simulink library "sm_car_testrig_utilities_lib"  (R2025a)
settings: Solver=VariableStepAuto  StartTime=0.0  StopTime=10.0  RelTol=1e-3
undefined symbols (not defined in the file): Maneuver, tire_radius, Vehicle, Visual, X, Y, Z
libraries: sm_lib x31, nesl_utility x18, fl_lib x3, $bdroot x3, Tire_Utilities x2, Surface_Profile_Axle2_KnC x2, simulink x2
(part 1 of 2)
Description:
  | Copyright 2026 The MathWorks, Inc.
settings Model: Creator=smiller  LastModifiedBy=smiller
settings OptimizationCC: ReuseModelBlockBuffer=off
settings ModelReferenceCC: EnableRefExpFcnMdlSchedulingChecks=on
settings RTWCC: GPUComputeCapability=3.5

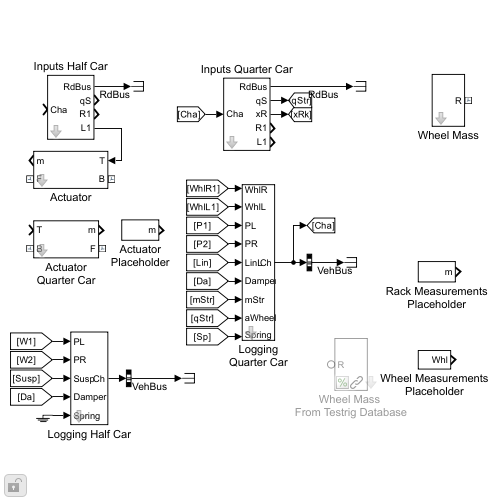
[thumbnail: Simulink's stored preview of the top-level diagram]
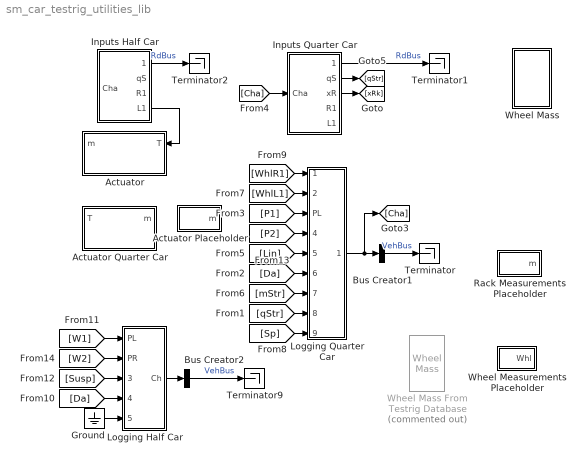
== system sm_car_testrig_utilities_lib ==
  Actuator : Subsystem  mask(KnC Actuator){tire_rad=tire_radius, xCPOffset=Maneuver.xCPOffset}
      mask prompts: tire_rad "Tire Radius (m)"; xCPOffset "xOffset from Contact Patch for force test (m)"
      mask help: Applies vertical motion to wheel center, permitting other DOFs to move freely. Can also apply force to wheel center, contact patch, and to a point behind the contact patch.
  Actuator Placeholder : Subsystem
  Actuator Quarter Car : Subsystem  mask{veh=Vehicle, xCPOffset=Maneuver.xCPOffset}
      mask prompts: veh "Vehicle (structure)"; xCPOffset "xOffset from Contact Patch for force test (m)"
      mask init:
      | tire_radii = sm_car_get_TireRadius(veh);
      | 
      | tire_radius = tire_radii(1);
      mask TypeOptions xCPOffset: Actuator/xCPOffset
  Bus Creator1 : BusCreator  Inputs=1
  Bus Creator2 : BusCreator  Inputs=1
  Ground : Ground
  Inputs Half Car : Subsystem  mask{popup_steering_input=On}
      mask prompts: popup_steering_input "Steering Input"
      mask init:
      | bh = gcb;
      | strIn = get_param(bh,'popup_steering_input');
      | set_param([bh '/Steering'], 'LabelModeActiveChoice',strIn);
      mask TypeOptions popup_steering_input: On | Off
  Inputs Quarter Car : Subsystem  mask{popup_steering_input=On}
      mask prompts: popup_steering_input "Steering Input"
      mask init:
      | bh = gcb;
      | strIn = get_param(bh,'popup_steering_input');
      | set_param([bh '/Steering'], 'LabelModeActiveChoice',strIn);
      mask TypeOptions popup_steering_input: On | Off
  Logging Quarter Car : Subsystem  mask(Logging Structure){}
      mask help: This subsystem takes logged signals and assembles them into a bus that has the same structure as the full vehicle model. This makes post-processing easier as the same scripts can be used.
      mask Display: disp(' ')
  Logging Half Car : Subsystem  mask(Logging Structure){}
      mask help: This subsystem takes logged signals and assembles them into a bus that has the same structure as the full vehicle model. This makes post-processing easier as the same scripts can be used.
      mask Display: disp(' ')
  Rack Measurements Placeholder : Subsystem
  Terminator{,1..2,9} (4 alike) : Terminator
  Wheel Mass : Subsystem  mask{tire_param=Vehicle.Chassis.TireA1.tirFile.Value}
      mask prompts: tire_param "Tire Parameters (structure)"
      mask init:
      | curblk = gcb;
      | 
      | %tireFile = evalin('base',get_param(curblk,'tire_param'));
      | %if(~contain(tire_param,'.tir'))
      | tireFile = tire_param;
      | if(contains(tireFile,'which'))
      |     tireFile = evalin('base',tireFile);
      | end
      | 
      | tirePar = simscape.multibody.tirread(tireFile);
      | 
      | tire_mass   = tirePar.INERTIA.MASS;
      | tire_radius = tirePar.DIMENSION.UNLOADED_RADIUS;
      | tire_width  = tirePar.DIMENSION.WIDTH;
  Wheel Mass From Testrig Database : $bdroot/Wheel Mass  Commented=on  tire_param=Vehicle.Chassis.TireA1
  Wheel Measurements Placeholder : Subsystem
  wires:
  [mStr] -> Logging Quarter Car/7(mStr)
  [Da] -> Logging Quarter Car/6(Damper)
  [Lin] -> Logging Quarter Car/5(LinL)
  [P2] -> Logging Quarter Car/4(PR)
  [qStr] -> Logging Quarter Car/8(aWheel)
  Inputs Quarter Car/2(qS) -> [qStr]
  Inputs Quarter Car/3(xR) -> [xRk]
  [Cha] -> Inputs Quarter Car/1(Cha)
  Logging Quarter Car/1(Ch) -> [Cha], Bus Creator1/1
  Bus Creator1/1 -> Terminator/1  "VehBus"
  Inputs Quarter Car/1(RdBus) -> Terminator1/1  "RdBus"
  [P1] -> Logging Quarter Car/3(PL)
  [WhlR1] -> Logging Quarter Car/1(WhlR)
  [WhlL1] -> Logging Quarter Car/2(WhlL)
  Inputs Half Car/1(RdBus) -> Terminator2/1  "RdBus"
  Logging Half Car/1(Ch) -> Bus Creator2/1
  Bus Creator2/1 -> Terminator9/1  "VehBus"
  [Sp] -> Logging Quarter Car/9(Spring)
  Ground/1 -> Logging Half Car/5(Spring)
  [Da] -> Logging Half Car/4(Damper)
  [Susp] -> Logging Half Car/3(Susp)
  [W2] -> Logging Half Car/2(PR)
  [W1] -> Logging Half Car/1(PL)
  Inputs Half Car/4(L1) -> Actuator/1(T)

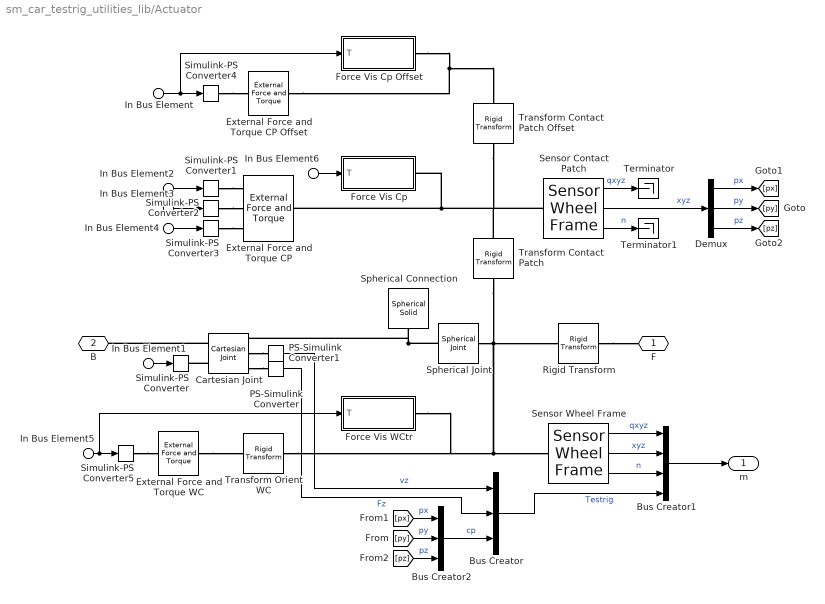
== system sm_car_testrig_utilities_lib/Actuator ==
  In Bus Element6 : Inport  PortName=T
  In Bus Element1 : Inport  PortName=T  Element=gz
  In Bus Element2 : Inport  PortName=T  Element=fcp.fx
  In Bus Element3 : Inport  PortName=T  Element=fcp.fy
  In Bus Element4 : Inport  PortName=T  Element=fcp.tz
  In Bus Element : Inport  PortName=T  Element=fcoy
  In Bus Element5 : Inport  PortName=T  Element=fwcx
  Bus Creator : BusCreator  Inputs=3
  Bus Creator1 : BusCreator  Inputs=4
  Bus Creator2 : BusCreator  Inputs=3
  Cartesian Joint : sm_lib/Joints/Cartesian Joint  JointMode=Normal  CompositeWrenchDir=FollowerOnBase  CompositeWrenchFrame=BaseFrame  SenseConstraintForce=off  SenseConstraintTorque=off  SenseTotalForce=off  SenseTotalTorque=off  PxPositionTargetSpecify=off  PxPositionTargetPriority=High  PxPositionTargetValue=0  PxPositionTargetValueUnits=m  PxVelocityTargetSpecify=off  PxVelocityTargetPriority=High  PxVelocityTargetValue=0  PxVelocityTargetValueUnits=m/s  PxEquilibriumPosition=0  PxEquilibriumPositionUnits=m  PxSpringStiffness=0  PxSpringStiffnessUnits=N/m  PxDampingCoefficient=0  PxDampingCoefficientUnits=N/(m/s)  PxLowerLimitSpecify=off  PxLowerLimitBound=-1  PxLowerLimitBoundUnits=m  PxLowerLimitStiffness=1e6  PxLowerLimitStiffnessUnits=N/m  PxLowerLimitDamping=1e3  PxLowerLimitDampingUnits=N/(m/s)  PxLowerLimitTransitionRegionWidth=1e-4  PxLowerLimitTransitionRegionWidthUnits=m  PxUpperLimitSpecify=off  PxUpperLimitBound=1  PxUpperLimitBoundUnits=m  PxUpperLimitStiffness=1e6  PxUpperLimitStiffnessUnits=N/m  PxUpperLimitDamping=1e3  PxUpperLimitDampingUnits=N/(m/s)  PxUpperLimitTransitionRegionWidth=1e-4  PxUpperLimitTransitionRegionWidthUnits=m  PxTorqueActuationMode=NoTorque  PxMotionActuationMode=ComputedMotion  PxSensePosition=off  PxSenseVelocity=off  PxSenseAcceleration=off  PxSenseTorqueForce=off  PxSenseLowerLimitTorqueForce=off  PxSenseUpperLimitTorqueForce=off  PyPositionTargetSpecify=off  PyPositionTargetPriority=High  PyPositionTargetValue=0  PyPositionTargetValueUnits=m  PyVelocityTargetSpecify=off  PyVelocityTargetPriority=High  PyVelocityTargetValue=0  PyVelocityTargetValueUnits=m/s  PyEquilibriumPosition=0  PyEquilibriumPositionUnits=m  PySpringStiffness=0  PySpringStiffnessUnits=N/m  PyDampingCoefficient=0  PyDampingCoefficientUnits=N/(m/s)  PyLowerLimitSpecify=off  PyLowerLimitBound=-1  PyLowerLimitBoundUnits=m  PyLowerLimitStiffness=1e6  PyLowerLimitStiffnessUnits=N/m  PyLowerLimitDamping=1e3  PyLowerLimitDampingUnits=N/(m/s)  PyLowerLimitTransitionRegionWidth=1e-4  PyLowerLimitTransitionRegionWidthUnits=m  PyUpperLimitSpecify=off  PyUpperLimitBound=1  PyUpperLimitBoundUnits=m  PyUpperLimitStiffness=1e6  PyUpperLimitStiffnessUnits=N/m  PyUpperLimitDamping=1e3  PyUpperLimitDampingUnits=N/(m/s)  PyUpperLimitTransitionRegionWidth=1e-4  PyUpperLimitTransitionRegionWidthUnits=m  PyTorqueActuationMode=NoTorque  PyMotionActuationMode=ComputedMotion  PySensePosition=off  PySenseVelocity=off  PySenseAcceleration=off  PySenseTorqueForce=off  PySenseLowerLimitTorqueForce=off  PySenseUpperLimitTorqueForce=off  PzPositionTargetSpecify=off  PzPositionTargetPriority=High  PzPositionTargetValue=0  PzPositionTargetValueUnits=m  PzVelocityTargetSpecify=off  PzVelocityTargetPriority=High  PzVelocityTargetValue=0  PzVelocityTargetValueUnits=m/s  PzEquilibriumPosition=0  PzEquilibriumPositionUnits=m  PzSpringStiffness=0  PzSpringStiffnessUnits=N/m  PzDampingCoefficient=0  PzDampingCoefficientUnits=N/(m/s)  PzLowerLimitSpecify=off  PzLowerLimitBound=-1  PzLowerLimitBoundUnits=m  PzLowerLimitStiffness=1e6  PzLowerLimitStiffnessUnits=N/m  PzLowerLimitDamping=1e3  PzLowerLimitDampingUnits=N/(m/s)  PzLowerLimitTransitionRegionWidth=1e-4  PzLowerLimitTransitionRegionWidthUnits=m  PzUpperLimitSpecify=off  PzUpperLimitBound=1  PzUpperLimitBoundUnits=m  PzUpperLimitStiffness=1e6  PzUpperLimitStiffnessUnits=N/m  PzUpperLimitDamping=1e3  PzUpperLimitDampingUnits=N/(m/s)  PzUpperLimitTransitionRegionWidth=1e-4  PzUpperLimitTransitionRegionWidthUnits=m  PzTorqueActuationMode=ComputedTorque  PzMotionActuationMode=InputMotion  PzSensePosition=off  PzSenseVelocity=on  PzSenseAcceleration=off  PzSenseTorqueForce=on  PzSenseLowerLimitTorqueForce=off  PzSenseUpperLimitTorqueForce=off
  Demux : Demux  Outputs=3
  External Force and Torque WC : sm_lib/Forces and Torques/External Force and Torque  EnableForceX=off  EnableForceY=on  EnableForceZ=off  EnableForce=off  ForceResolutionFrame=World  EnableTorqueX=off  EnableTorqueY=off  EnableTorqueZ=off  EnableTorque=off  TorqueResolutionFrame=World
  External Force and Torque CP : sm_lib/Forces and Torques/External Force and Torque  EnableForceX=on  EnableForceY=on  EnableForceZ=off  EnableForce=off  ForceResolutionFrame=World  EnableTorqueX=off  EnableTorqueY=off  EnableTorqueZ=on  EnableTorque=off  TorqueResolutionFrame=World
  External Force and Torque CP Offset : sm_lib/Forces and Torques/External Force and Torque  EnableForceX=off  EnableForceY=on  EnableForceZ=off  EnableForce=off  ForceResolutionFrame=World  EnableTorqueX=off  EnableTorqueY=off  EnableTorqueZ=off  EnableTorque=off  TorqueResolutionFrame=World
  Force Vis Cp : Subsystem  mask(Force and Torque Visualization){fcyl_opc=0.2, fcyl_clr=[1 0 0], fcyl_rad=0.02, fcyl_len=0.8, tcyl_rad=0.25, tcyl_clrn=[0.3922 0.8314 0.07451], max_fx=max(Maneuver.PostL1.fx.Value), max_fy=max(Maneuver.PostL1.fy.Value), max_tz=max(Maneuver.PostL1.tz.Value)}
      mask prompts: fcyl_opc "Opacity (0-1)"; fcyl_clr "Color [RGB]"; fcyl_rad "Radius (m)"; fcyl_len "Max Length (m)"; tcyl_rad "Max Radius (m)"; tcyl_clrn "Color for negative [RGB]"; max_fx "Max Fx (N)"; max_fy "Max Fy (N)"; max_tz "Max Tz (N)"
      mask help: Provides visual element for force and torque. Force visualization extends in direction along which force is applied. Torque visualization uses alternate color for opposite sign.
      mask DialogControl cont_fcyl Prompt: Force Cylinders
      mask DialogControl cont_trqcyl Prompt: Torque Cylinders
      mask DialogControl cont_fmax Prompt: Force/Torque Magnitudes
  Force Vis Cp Offset : Subsystem  mask(Force Visualization){fcyl_opc=0.2, fcyl_clr=[1 0 0], fcyl_rad=0.02, fcyl_len=0.8, tcyl_rad=0.25, tcyl_clrn=[0.3922 0.8314 0.07451], fy_max=max(Maneuver.PostL1.fcoy.Value)}
      mask prompts: fcyl_opc "Opacity (0-1)"; fcyl_clr "Color [RGB]"; fcyl_rad "Radius (m)"; fcyl_len "Max Length (m)"; tcyl_rad "Max Radius (m)"; tcyl_clrn "Color for negative [RGB]"; fy_max "Max Fx (N)"
      mask help: Provides visual element for force. Extends in direction along which force is applied.
      mask DialogControl cont_fcyl Prompt: Force Cylinders
      mask DialogControl cont_trqcyl Prompt: Torque Cylinders
      mask DialogControl cont_fmx Prompt: Force Magnitudes
  Force Vis WCtr : Subsystem  mask(Force Visualization){fcyl_opc=0.2, fcyl_clr=[1 0 0], fcyl_rad=0.02, fcyl_len=0.8, max_fx=max(Maneuver.PostL1.fwcx.Value)}
      mask prompts: fcyl_opc "Opacity (0-1)"; fcyl_clr "Color [RGB]"; fcyl_rad "Radius (m)"; fcyl_len "Max Length (m)"; max_fx "Max Fx(N)"
      mask help: Provides visual element for force. Extends in direction along which force is applied.
      mask DialogControl cont_fcyl Prompt: Force Cylinders
      mask DialogControl cont_fmax Prompt: Force Magnitudes
  PS-Simulink Converter : nesl_utility/PS-Simulink Converter  PhysicalDomain=network_engine_domain  SubClassName=ps_output  LeftPortType=input  RightPortType=output  PseudoPeriodic=off  Frequencies=[]  VectorFormat=1-D array  Unit=1  AffineConversion=off
  PS-Simulink Converter1 : nesl_utility/PS-Simulink Converter  PhysicalDomain=network_engine_domain  SubClassName=ps_output  LeftPortType=input  RightPortType=output  PseudoPeriodic=off  Frequencies=[]  VectorFormat=1-D array  Unit=1  AffineConversion=off
  Rigid Transform : sm_lib/Frames and Transforms/Rigid Transform  RotationMethod=StandardAxis  FollAlignAxisA=+X  BaseAlignAxisA=+Y  FollAlignAxisB=+Y  BaseAlignAxisB=+Z  RotationStandardAxis=+X  RotationAngle=-90  RotationAngleUnits=deg  RotationArbitraryAxis=[0 0 1]  RotationSequenceAxes=FollowerAxes  RotationSequence=XYX  RotationSequenceAngles=[0 0 0]  RotationSequenceAnglesUnits=deg  RotationMatrix=[1 0 0; 0 1 0; 0 0 1]  Quaternion=[1 0 0 0]  TranslationMethod=None  TranslationCartesianOffset=[0 0 0]  TranslationCartesianOffsetUnits=m  TranslationStandardAxis=+Z  TranslationStandardOffset=0  TranslationStandardOffsetUnits=m  TranslationROffset=0  TranslationROffsetUnits=m  TranslationThetaOffset=0  TranslationThetaOffsetUnits=deg  TranslationZOffset=0  TranslationZOffsetUnits=m
  Sensor Contact Patch : Tire_Utilities/Sensor Wheel Frame  SystemSampleTime=-1  VariantActivationTime=update diagram  EmptyChoice=off  PassThrough=off  PassThroughVariantControl=(default)  EmptyChoiceVariantControl=(default)  AllowFlexibleInterface=on  Latency=0  AutoFrameSizeCalculation=off
  Sensor Wheel Frame : Tire_Utilities/Sensor Wheel Frame  SystemSampleTime=-1  VariantActivationTime=update diagram  EmptyChoice=off  PassThrough=off  PassThroughVariantControl=(default)  EmptyChoiceVariantControl=(default)  AllowFlexibleInterface=on  Latency=0  AutoFrameSizeCalculation=off
  Simulink-PS Converter : nesl_utility/Simulink-PS Converter  PhysicalDomain=network_engine_domain  SubClassName=ps_input  LeftPortType=input  RightPortType=output  PseudoPeriodic=off  Frequencies=[]  NoiseDistribution=none  NoiseParameters=[]  Unit=m  AffineConversion=off  FilteringAndDerivatives=filter  SimscapeFilterOrder=2  InputFilterTimeConstant=0.1  UdotUserProvided=0
  Simulink-PS Converter{1..5} (5 alike) : nesl_utility/Simulink-PS Converter  PhysicalDomain=network_engine_domain  SubClassName=ps_input  LeftPortType=input  RightPortType=output  PseudoPeriodic=off  Frequencies=[]  NoiseDistribution=none  NoiseParameters=[]  Unit=1  AffineConversion=off  FilteringAndDerivatives=provide  SimscapeFilterOrder=1  InputFilterTimeConstant=0.001  UdotUserProvided=0
  Spherical Connection : sm_lib/Body Elements/Spherical Solid  SphereRadius=Visual.hp.rad*1.5  SphereRadiusUnits=m  ExportEntireGeometry=off  InertiaType=CalculateFromGeometry  BasedOnType=Density  Density=1000  DensityUnits=kg/m^3  Mass=1  MassUnits=kg  CenterOfMass=[0 0 0]  CenterOfMassUnits=m  MomentsOfInertia=[1 1 1]  MomentsOfInertiaUnits=kg*m^2  ProductsOfInertia=[0 0 0]  ProductsOfInertiaUnits=kg*m^2  GraphicType=FromGeometry  MarkerShape=Sphere  MarkerSize=10  GraphicVisPropType=SimpleVisualProperties  GraphicDiffuseColor=[0.2 0.2 1.0]  GraphicOpacity=0.5  GraphicSpecularColor=[0.5 0.5 0.5 1.0]  GraphicAmbientColor=[0.15 0.15 0.15 1.0]  GraphicEmissiveColor=[0.0 0.0 0.0 1.0]  GraphicShininess=75  DoExposeReferenceFrame=on  SerializedFrames=<Frames/>
  Spherical Joint : sm_lib/Joints/Spherical Joint  JointMode=Normal  CompositeWrenchDir=FollowerOnBase  CompositeWrenchFrame=BaseFrame  SenseConstraintForce=off  SenseConstraintTorque=off  SenseTotalForce=off  SenseTotalTorque=off  PositionTargetSpecify=off  PositionTargetPriority=High  PositionTargetRotationMethod=None  PositionTargetFollAlignAxisA=+X  PositionTargetBaseAlignAxisA=+Y  PositionTargetFollAlignAxisB=+Y  PositionTargetBaseAlignAxisB=+Z  PositionTargetRotationStandardAxis=+Z  PositionTargetRotationAngle=0.0  PositionTargetRotationAngleUnits=deg  PositionTargetRotationArbitraryAxis=[0 0 1]  PositionTargetRotationSequenceAxes=FollowerAxes  PositionTargetRotationSequence=XYX  PositionTargetRotationSequenceAngles=[0 0 0]  PositionTargetRotationSequenceAnglesUnits=deg  PositionTargetRotationMatrix=[1 0 0; 0 1 0; 0 0 1]  PositionTargetQuaternion=[1 0 0 0]  VelocityTargetSpecify=off  VelocityTargetPriority=High  VelocityTargetValue=[0 0 0]  VelocityTargetValueUnits=deg/s  VelocityTargetInFollowerFrame=on  EqPosRotationMethod=None  EqPosFollAlignAxisA=+X  EqPosBaseAlignAxisA=+Y  EqPosFollAlignAxisB=+Y  EqPosBaseAlignAxisB=+Z  EqPosRotationStandardAxis=+Z  EqPosRotationAngle=0.0  EqPosRotationAngleUnits=deg  EqPosRotationArbitraryAxis=[0 0 1]  EqPosRotationSequenceAxes=FollowerAxes  EqPosRotationSequence=XYX  EqPosRotationSequenceAngles=[0 0 0]  EqPosRotationSequenceAnglesUnits=deg  EqPosRotationMatrix=[1 0 0; 0 1 0; 0 0 1]  EqPosQuaternion=[1 0 0 0]  SpringStiffness=0  SpringStiffnessUnits=N*m/deg  DampingCoefficient=0  DampingCoefficientUnits=N*m/(deg/s)  LowerLimitSpecify=off  LowerLimitBound=15  LowerLimitBoundUnits=deg  LowerLimitStiffness=1e4  LowerLimitStiffnessUnits=N*m/deg  LowerLimitDamping=10  LowerLimitDampingUnits=N*m/(deg/s)  LowerLimitTransitionRegionWidth=0.1  LowerLimitTransitionRegionWidthUnits=deg  UpperLimitSpecify=off  UpperLimitBound=45  UpperLimitBoundUnits=deg  UpperLimitStiffness=1e4  UpperLimitStiffnessUnits=N*m/deg  UpperLimitDamping=10  UpperLimitDampingUnits=N*m/(deg/s)  UpperLimitTransitionRegionWidth=0.1  UpperLimitTransitionRegionWidthUnits=deg  TorqueActuationMode=NoTorque  ActuateTorqueX=off  ActuateTorqueY=off  ActuateTorqueZ=off  ActuateTorque=off  ActuationFrame=BaseFrame  SensePosition=off  SenseVelocityX=off  SenseVelocityY=off  SenseVelocityZ=off  SenseVelocity=off  SenseAccelerationX=off  SenseAccelerationY=off  SenseAccelerationZ=off  SenseAcceleration=off  SenseLowerLimitTorqueMag=off  SenseUpperLimitTorqueMag=off  SensingFrame=BaseFrame
  Terminator : Terminator
  Terminator1 : Terminator
  Transform Contact Patch : sm_lib/Frames and Transforms/Rigid Transform  RotationMethod=None  FollAlignAxisA=+X  BaseAlignAxisA=+Y  FollAlignAxisB=+Y  BaseAlignAxisB=+Z  RotationStandardAxis=+X  RotationAngle=90  RotationAngleUnits=deg  RotationArbitraryAxis=[0 0 1]  RotationSequenceAxes=FollowerAxes  RotationSequence=XYX  RotationSequenceAngles=[0 0 0]  RotationSequenceAnglesUnits=deg  RotationMatrix=[1 0 0; 0 1 0; 0 0 1]  Quaternion=[1 0 0 0]  TranslationMethod=Cartesian  TranslationCartesianOffset=[0 0 -tire_rad]  TranslationCartesianOffsetUnits=m  TranslationStandardAxis=+Z  TranslationStandardOffset=0  TranslationStandardOffsetUnits=m  TranslationROffset=0  TranslationROffsetUnits=m  TranslationThetaOffset=0  TranslationThetaOffsetUnits=deg  TranslationZOffset=0  TranslationZOffsetUnits=m
  Transform Contact Patch Offset : sm_lib/Frames and Transforms/Rigid Transform  RotationMethod=None  FollAlignAxisA=+X  BaseAlignAxisA=+Y  FollAlignAxisB=+Y  BaseAlignAxisB=+Z  RotationStandardAxis=+X  RotationAngle=90  RotationAngleUnits=deg  RotationArbitraryAxis=[0 0 1]  RotationSequenceAxes=FollowerAxes  RotationSequence=XYX  RotationSequenceAngles=[0 0 0]  RotationSequenceAnglesUnits=deg  RotationMatrix=[1 0 0; 0 1 0; 0 0 1]  Quaternion=[1 0 0 0]  TranslationMethod=Cartesian  TranslationCartesianOffset=[xCPOffset 0 0]  TranslationCartesianOffsetUnits=m  TranslationStandardAxis=+Z  TranslationStandardOffset=0  TranslationStandardOffsetUnits=m  TranslationROffset=0  TranslationROffsetUnits=m  TranslationThetaOffset=0  TranslationThetaOffsetUnits=deg  TranslationZOffset=0  TranslationZOffsetUnits=m
  Transform Orient WC : sm_lib/Frames and Transforms/Rigid Transform  RotationMethod=StandardAxis  FollAlignAxisA=+X  BaseAlignAxisA=+Y  FollAlignAxisB=+Y  BaseAlignAxisB=+Z  RotationStandardAxis=+X  RotationAngle=90  RotationAngleUnits=deg  RotationArbitraryAxis=[0 0 1]  RotationSequenceAxes=FollowerAxes  RotationSequence=XYX  RotationSequenceAngles=[0 0 0]  RotationSequenceAnglesUnits=deg  RotationMatrix=[1 0 0; 0 1 0; 0 0 1]  Quaternion=[1 0 0 0]  TranslationMethod=Cartesian  TranslationCartesianOffset=[0 0 0]  TranslationCartesianOffsetUnits=m  TranslationStandardAxis=+Z  TranslationStandardOffset=0  TranslationStandardOffsetUnits=m  TranslationROffset=0  TranslationROffsetUnits=m  TranslationThetaOffset=0  TranslationThetaOffsetUnits=deg  TranslationZOffset=0  TranslationZOffsetUnits=m
  F : PMIOPort  Side=Right
  B : PMIOPort  Port=2  Side=Left
  m : Outport  VectorParamsAs1DForOutWhenUnconnected=off
  wires:
  In Bus Element1/1 -> Simulink-PS Converter/1
  In Bus Element3/1 -> Simulink-PS Converter2/1
  Demux/2 -> [py]  "py"
  In Bus Element4/1 -> Simulink-PS Converter3/1
  Sensor Contact Patch/2 -> Demux/1  "xyz"
  Sensor Contact Patch/1 -> Terminator/1  "qxyz"
  In Bus Element2/1 -> Simulink-PS Converter1/1
  Sensor Contact Patch/3 -> Terminator1/1  "n"
  Sensor Wheel Frame/2 -> Bus Creator1/2  "xyz"
  Sensor Wheel Frame/1 -> Bus Creator1/1  "qxyz"
  Bus Creator/1 -> Bus Creator1/4  "Testrig"
  Bus Creator1/1 -> m/1
  PS-Simulink Converter/1 -> Bus Creator/2  "Fz"
  Sensor Wheel Frame/3 -> Bus Creator1/3  "n"
  [py] -> Bus Creator2/2  "py"
  Demux/1 -> [px]  "px"
  [px] -> Bus Creator2/1  "px"
  In Bus Element/1 -> Force Vis Cp Offset/1(T), Simulink-PS Converter4/1
  In Bus Element5/1 -> Force Vis WCtr/1(T), Simulink-PS Converter5/1
  In Bus Element6/1 -> Force Vis Cp/1(T)
  PS-Simulink Converter1/1 -> Bus Creator/1  "vz"
  Demux/3 -> [pz]  "pz"
  [pz] -> Bus Creator2/3  "pz"
  Bus Creator2/1 -> Bus Creator/3  "cp"
  connections:
  Rigid Transform/RConn1 -- F/RConn1
  Spherical Joint/LConn1 -- Cartesian Joint/RConn1 -- Spherical Connection/RConn1
  Spherical Joint/RConn1 -- Force Vis WCtr/RConn1 -- Transform Orient WC/LConn1 -- Sensor Wheel Frame/LConn1 -- Transform Contact Patch/LConn1 -- Rigid Transform/LConn1
  Cartesian Joint/LConn1 -- B/RConn1
  Cartesian Joint/LConn2 -- Simulink-PS Converter/RConn1
  Cartesian Joint/RConn3 -- PS-Simulink Converter/LConn1
  Transform Contact Patch Offset/LConn1 -- Sensor Contact Patch/LConn1 -- Transform Contact Patch/RConn1 -- External Force and Torque CP/RConn1 -- Force Vis Cp/RConn1
  Simulink-PS Converter1/RConn1 -- External Force and Torque CP/LConn1
  Simulink-PS Converter3/RConn1 -- External Force and Torque CP/LConn3
  Simulink-PS Converter2/RConn1 -- External Force and Torque CP/LConn2
  External Force and Torque CP Offset/RConn1 -- Force Vis Cp Offset/RConn1 -- Transform Contact Patch Offset/RConn1
  Simulink-PS Converter4/RConn1 -- External Force and Torque CP Offset/LConn1
  Simulink-PS Converter5/RConn1 -- External Force and Torque WC/LConn1
  External Force and Torque WC/RConn1 -- Transform Orient WC/RConn1
  Cartesian Joint/RConn2 -- PS-Simulink Converter1/LConn1

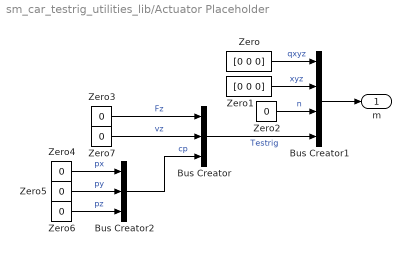
== system sm_car_testrig_utilities_lib/Actuator Placeholder ==
  Bus Creator : BusCreator  Inputs=3
  Bus Creator1 : BusCreator  Inputs=4
  Bus Creator2 : BusCreator  Inputs=3
  Zero : Constant  Value=[0 0 0]  OutDataTypeStr=Inherit: Inherit via back propagation
  Zero1 : Constant  Value=[0 0 0]  OutDataTypeStr=Inherit: Inherit via back propagation
  Zero{2..7} (6 alike) : Constant  Value=0  OutDataTypeStr=Inherit: Inherit via back propagation
  m : Outport
  wires:
  Zero4/1 -> Bus Creator2/1  "px"
  Zero1/1 -> Bus Creator1/2  "xyz"
  Zero2/1 -> Bus Creator1/3  "n"
  Zero/1 -> Bus Creator1/1  "qxyz"
  Zero3/1 -> Bus Creator/1  "Fz"
  Zero5/1 -> Bus Creator2/2  "py"
  Bus Creator/1 -> Bus Creator1/4  "Testrig"
  Bus Creator1/1 -> m/1
  Zero6/1 -> Bus Creator2/3  "pz"
  Bus Creator2/1 -> Bus Creator/3  "cp"
  Zero7/1 -> Bus Creator/2  "vz"

== system sm_car_testrig_utilities_lib/Actuator Quarter Car ==
  T : Inport
  Actuator : $bdroot/Actuator  tire_rad=tire_radius  xCPOffset=xCPOffset
  F : PMIOPort  Side=Right
  B : PMIOPort  Port=2  Side=Left
  m : Outport
  wires:
  Actuator/1 -> m/1
  T/1 -> Actuator/1
  connections:
  Actuator/LConn1 -- B/RConn1
  Actuator/RConn1 -- F/RConn1

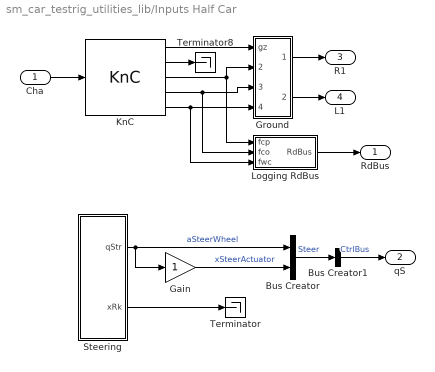
== system sm_car_testrig_utilities_lib/Inputs Half Car ==
  Cha : Inport
  Bus Creator : BusCreator  Inputs=2
  Bus Creator1 : BusCreator  Inputs=1
  Gain : Gain
  Ground : Subsystem
  KnC : Surface_Profile_Axle2_KnC/KnC  SystemSampleTime=-1  VariantControl=KnC  VariantActivationTime=update diagram  EmptyChoice=off  PassThrough=off  PassThroughVariantControl=(default)  EmptyChoiceVariantControl=(default)  AllowFlexibleInterface=on  Latency=0  AutoFrameSizeCalculation=off
  Logging RdBus : Subsystem
  Steering : Subsystem  Variant=on  VariantControlMode=label  VariantControl=Choice  LabelModeActiveChoice=On
  Terminator : Terminator
  Terminator8 : Terminator
  RdBus : Outport
  qS : Outport  Port=2
  R1 : Outport  Port=3
  L1 : Outport  Port=4
  wires:
  Logging RdBus/1(RdBus) -> RdBus/1
  Steering/2(xRk) -> Terminator/1
  Steering/1(qStr) -> Gain/1, Bus Creator/1  "aSteerWheel"
  Ground/1(R1) -> R1/1
  Cha/1 -> KnC/1
  KnC/1 -> Ground/1(gz)
  Ground/2(L1) -> L1/1
  KnC/3 -> Logging RdBus/1(fcp), Ground/2(fcp)
  KnC/2 -> Terminator8/1
  Bus Creator1/1 -> qS/1  "CtrlBus"
  Bus Creator/1 -> Bus Creator1/1  "Steer"
  KnC/4 -> Logging RdBus/2(fco), Ground/3(fco)
  KnC/5 -> Logging RdBus/3(fwc), Ground/4(fwc)
  Gain/1 -> Bus Creator/2  "xSteerActuator"

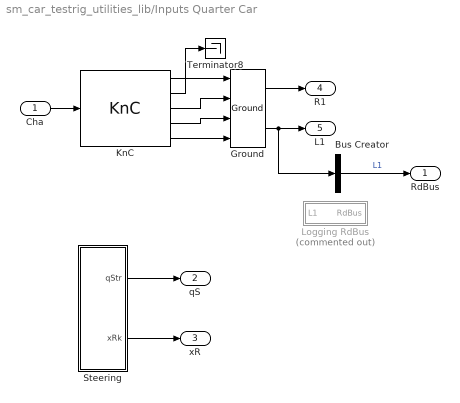
== system sm_car_testrig_utilities_lib/Inputs Quarter Car ==
  Cha : Inport
  Bus Creator : BusCreator  Inputs=1
  Ground : $bdroot/Inputs Half Car/Ground  SystemSampleTime=-1  VariantActivationTime=update diagram  EmptyChoice=off  PassThrough=off  PassThroughVariantControl=(default)  EmptyChoiceVariantControl=(default)  AllowFlexibleInterface=on  Latency=0  AutoFrameSizeCalculation=off
  KnC : Surface_Profile_Axle2_KnC/KnC  SystemSampleTime=-1  VariantControl=KnC  VariantActivationTime=update diagram  EmptyChoice=off  PassThrough=off  PassThroughVariantControl=(default)  EmptyChoiceVariantControl=(default)  AllowFlexibleInterface=on  Latency=0  AutoFrameSizeCalculation=off
  Logging RdBus : Subsystem  Commented=on
  Steering : Subsystem  Variant=on  VariantControlMode=label  VariantControl=Choice  LabelModeActiveChoice=On
  Terminator8 : Terminator
  RdBus : Outport
  qS : Outport  Port=2
  xR : Outport  Port=3
  R1 : Outport  Port=4
  L1 : Outport  Port=5
  wires:
  KnC/2 -> Terminator8/1
  KnC/3 -> Ground/2
  KnC/1 -> Ground/1
  Cha/1 -> KnC/1
  Ground/1 -> R1/1
  Steering/1(qStr) -> qS/1
  Steering/2(xRk) -> xR/1
  Ground/2 -> Bus Creator/1, L1/1
  KnC/4 -> Ground/3
  KnC/5 -> Ground/4
  Bus Creator/1 -> RdBus/1  "L1"

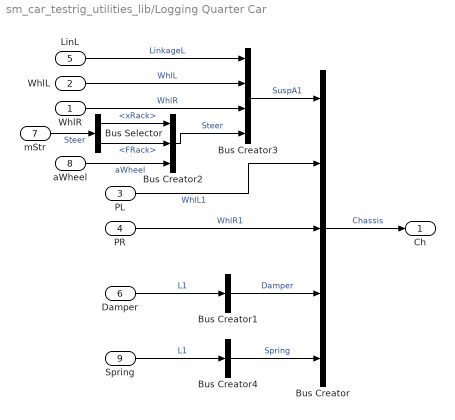
== system sm_car_testrig_utilities_lib/Logging Quarter Car ==
  WhlR : Inport
  WhlL : Inport  Port=2
  PL : Inport  Port=3
  PR : Inport  Port=4
  LinL : Inport  Port=5
  Damper : Inport  Port=6
  mStr : Inport  Port=7
  aWheel : Inport  Port=8
  Spring : Inport  Port=9
  Bus Creator : BusCreator  Inputs=5
  Bus Creator1 : BusCreator  Inputs=1
  Bus Creator2 : BusCreator  Inputs=3
  Bus Creator3 : BusCreator  Inputs=4
  Bus Creator4 : BusCreator  Inputs=1
  Bus Selector : BusSelector  OutputSignals=xRack,FRack
  Ch : Outport
  wires:
  Bus Selector/2 -> Bus Creator2/2  "<FRack>"
  Bus Selector/1 -> Bus Creator2/1  "<xRack>"
  mStr/1 -> Bus Selector/1  "Steer"
  PR/1 -> Bus Creator/3  "WhlR1"
  WhlR/1 -> Bus Creator3/3  "WhlR"
  PL/1 -> Bus Creator/2  "WhlL1"
  Bus Creator3/1 -> Bus Creator/1  "SuspA1"
  Bus Creator/1 -> Ch/1  "Chassis"
  LinL/1 -> Bus Creator3/1  "LinkageL"
  WhlL/1 -> Bus Creator3/2  "WhlL"
  Damper/1 -> Bus Creator1/1  "L1"
  Bus Creator2/1 -> Bus Creator3/4  "Steer"
  Bus Creator1/1 -> Bus Creator/4  "Damper"
  aWheel/1 -> Bus Creator2/3  "aWheel"
  Spring/1 -> Bus Creator4/1  "L1"
  Bus Creator4/1 -> Bus Creator/5  "Spring"

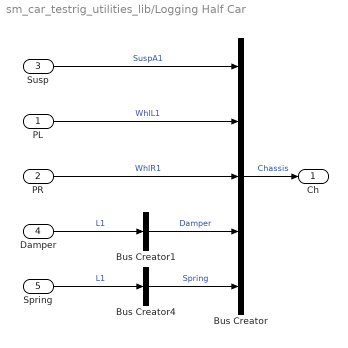
== system sm_car_testrig_utilities_lib/Logging Half Car ==
  PL : Inport
  PR : Inport  Port=2
  Susp : Inport  Port=3
  Damper : Inport  Port=4
  Spring : Inport  Port=5
  Bus Creator : BusCreator  Inputs=5
  Bus Creator1 : BusCreator  Inputs=1
  Bus Creator4 : BusCreator  Inputs=1
  Ch : Outport
  wires:
  PR/1 -> Bus Creator/3  "WhlR1"
  Bus Creator4/1 -> Bus Creator/5  "Spring"
  Spring/1 -> Bus Creator4/1  "L1"
  Bus Creator1/1 -> Bus Creator/4  "Damper"
  Damper/1 -> Bus Creator1/1  "L1"
  Bus Creator/1 -> Ch/1  "Chassis"
  Susp/1 -> Bus Creator/1  "SuspA1"
  PL/1 -> Bus Creator/2  "WhlL1"

== system sm_car_testrig_utilities_lib/Rack Measurements Placeholder ==
  Bus Creator2 : BusCreator  Inputs=2
  Zero3 : Constant  Value=0  OutDataTypeStr=Inherit: Inherit via back propagation
  Zero4 : Constant  Value=0  OutDataTypeStr=Inherit: Inherit via back propagation
  m : Outport
  wires:
  Bus Creator2/1 -> m/1
  Zero4/1 -> Bus Creator2/2  "FRack"
  Zero3/1 -> Bus Creator2/1  "xRack"

== system sm_car_testrig_utilities_lib/Wheel Mass ==
  Wheel Mass : sm_lib/Body Elements/Cylindrical Solid  CylinderRadius=tire_radius  CylinderRadiusUnits=m  CylinderLength=tire_width  CylinderLengthUnits=m  ExportEntireGeometry=off  InertiaType=CalculateFromGeometry  BasedOnType=Mass  Density=1000  DensityUnits=kg/m^3  Mass=tire_mass  MassUnits=kg  CenterOfMass=[0 0 0]  CenterOfMassUnits=m  MomentsOfInertia=[1 1 1]  MomentsOfInertiaUnits=kg*m^2  ProductsOfInertia=[0 0 0]  ProductsOfInertiaUnits=kg*m^2  GraphicType=FromGeometry  MarkerShape=Sphere  MarkerSize=10  GraphicVisPropType=SimpleVisualProperties  GraphicDiffuseColor=[0.5 0.5 0.5]  GraphicOpacity=0.3  GraphicSpecularColor=[0.5 0.5 0.5 1.0]  GraphicAmbientColor=[0.15 0.15 0.15 1.0]  GraphicEmissiveColor=[0.0 0.0 0.0 1.0]  GraphicShininess=75  DoExposeReferenceFrame=on  SerializedFrames=<Frames/>
  R : PMIOPort  Side=Right
  connections:
  Wheel Mass/RConn1 -- R/RConn1

== system sm_car_testrig_utilities_lib/Wheel Measurements Placeholder ==
  Bus Creator : BusCreator  Inputs=4
  Zero{1..4} (4 alike) : Constant  Value=0  OutDataTypeStr=Inherit: Inherit via back propagation
  Whl : Outport
  wires:
  Zero4/1 -> Bus Creator/4  "aCamberX"
  Bus Creator/1 -> Whl/1  "Whl"
  Zero3/1 -> Bus Creator/3  "aToeX"
  Zero1/1 -> Bus Creator/1  "aToe"
  Zero2/1 -> Bus Creator/2  "aCamber"

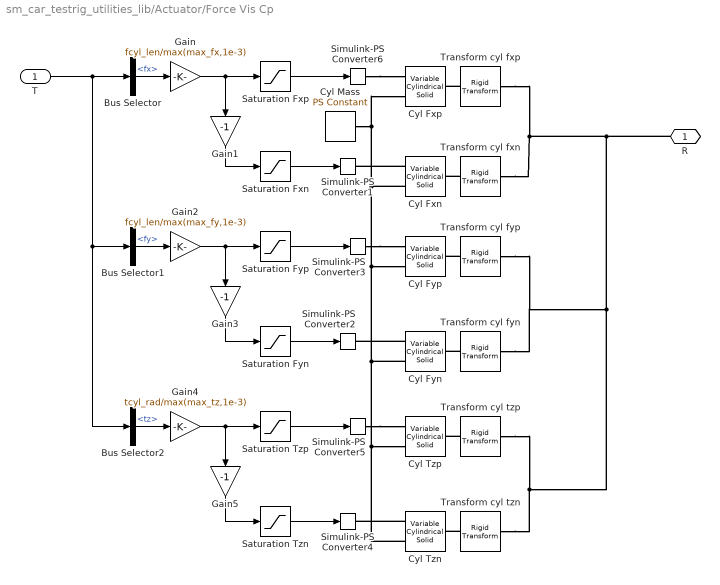
== system sm_car_testrig_utilities_lib/Actuator/Force Vis Cp ==
  T : Inport
  Bus Selector : BusSelector  OutputSignals=fcp.fx
  Bus Selector1 : BusSelector  OutputSignals=fcp.fy
  Bus Selector2 : BusSelector  OutputSignals=fcp.tz
  Cyl Fxn : sm_lib/Body Elements/Variable Mass/Variable Cylindrical Solid  RadiusType=Constant  Radius=fcyl_rad  RadiusUnits=m  LengthType=ProvidedByInput  Length=1e-3  LengthUnits=m  MassType=ProvidedByInput  Density=1000  DensityUnits=kg/m^3  SenseRadius=off  SenseLength=off  SenseMass=off  SenseCenterOfMass=off  SenseInertiaMatrix=off  GraphicType=FromGeometry  MarkerShape=Sphere  MarkerSize=10  GraphicVisPropType=SimpleVisualProperties  GraphicDiffuseColor=fcyl_clr  GraphicOpacity=fcyl_opc  GraphicSpecularColor=[0.5 0.5 0.5 1.0]  GraphicAmbientColor=[0.15 0.15 0.15 1.0]  GraphicEmissiveColor=[0.0 0.0 0.0 1.0]  GraphicShininess=75
  Cyl Fxp : sm_lib/Body Elements/Variable Mass/Variable Cylindrical Solid  RadiusType=Constant  Radius=fcyl_rad  RadiusUnits=m  LengthType=ProvidedByInput  Length=1e-3  LengthUnits=m  MassType=ProvidedByInput  Density=1000  DensityUnits=kg/m^3  SenseRadius=off  SenseLength=off  SenseMass=off  SenseCenterOfMass=off  SenseInertiaMatrix=off  GraphicType=FromGeometry  MarkerShape=Sphere  MarkerSize=10  GraphicVisPropType=SimpleVisualProperties  GraphicDiffuseColor=fcyl_clr  GraphicOpacity=fcyl_opc  GraphicSpecularColor=[0.5 0.5 0.5 1.0]  GraphicAmbientColor=[0.15 0.15 0.15 1.0]  GraphicEmissiveColor=[0.0 0.0 0.0 1.0]  GraphicShininess=75
  Cyl Fyn : sm_lib/Body Elements/Variable Mass/Variable Cylindrical Solid  RadiusType=Constant  Radius=fcyl_rad  RadiusUnits=m  LengthType=ProvidedByInput  Length=1e-3  LengthUnits=m  MassType=ProvidedByInput  Density=1000  DensityUnits=kg/m^3  SenseRadius=off  SenseLength=off  SenseMass=off  SenseCenterOfMass=off  SenseInertiaMatrix=off  GraphicType=FromGeometry  MarkerShape=Sphere  MarkerSize=10  GraphicVisPropType=SimpleVisualProperties  GraphicDiffuseColor=fcyl_clr  GraphicOpacity=fcyl_opc  GraphicSpecularColor=[0.5 0.5 0.5 1.0]  GraphicAmbientColor=[0.15 0.15 0.15 1.0]  GraphicEmissiveColor=[0.0 0.0 0.0 1.0]  GraphicShininess=75
  Cyl Fyp : sm_lib/Body Elements/Variable Mass/Variable Cylindrical Solid  RadiusType=Constant  Radius=fcyl_rad  RadiusUnits=m  LengthType=ProvidedByInput  Length=1e-3  LengthUnits=m  MassType=ProvidedByInput  Density=1000  DensityUnits=kg/m^3  SenseRadius=off  SenseLength=off  SenseMass=off  SenseCenterOfMass=off  SenseInertiaMatrix=off  GraphicType=FromGeometry  MarkerShape=Sphere  MarkerSize=10  GraphicVisPropType=SimpleVisualProperties  GraphicDiffuseColor=fcyl_clr  GraphicOpacity=fcyl_opc  GraphicSpecularColor=[0.5 0.5 0.5 1.0]  GraphicAmbientColor=[0.15 0.15 0.15 1.0]  GraphicEmissiveColor=[0.0 0.0 0.0 1.0]  GraphicShininess=75
  Cyl Mass : fl_lib/Physical Signals/Sources/PS Constant  constant=1e-3
  Cyl Tzn : sm_lib/Body Elements/Variable Mass/Variable Cylindrical Solid  RadiusType=ProvidedByInput  Radius=fcyl_rad  RadiusUnits=m  LengthType=Constant  Length=1e-3  LengthUnits=m  MassType=ProvidedByInput  Density=1000  DensityUnits=kg/m^3  SenseRadius=off  SenseLength=off  SenseMass=off  SenseCenterOfMass=off  SenseInertiaMatrix=off  GraphicType=FromGeometry  MarkerShape=Sphere  MarkerSize=10  GraphicVisPropType=SimpleVisualProperties  GraphicDiffuseColor=tcyl_clrn  GraphicOpacity=fcyl_opc  GraphicSpecularColor=[0.5 0.5 0.5 1.0]  GraphicAmbientColor=[0.15 0.15 0.15 1.0]  GraphicEmissiveColor=[0.0 0.0 0.0 1.0]  GraphicShininess=75
  Cyl Tzp : sm_lib/Body Elements/Variable Mass/Variable Cylindrical Solid  RadiusType=ProvidedByInput  Radius=fcyl_rad  RadiusUnits=m  LengthType=Constant  Length=1e-3  LengthUnits=m  MassType=ProvidedByInput  Density=1000  DensityUnits=kg/m^3  SenseRadius=off  SenseLength=off  SenseMass=off  SenseCenterOfMass=off  SenseInertiaMatrix=off  GraphicType=FromGeometry  MarkerShape=Sphere  MarkerSize=10  GraphicVisPropType=SimpleVisualProperties  GraphicDiffuseColor=fcyl_clr  GraphicOpacity=fcyl_opc  GraphicSpecularColor=[0.5 0.5 0.5 1.0]  GraphicAmbientColor=[0.15 0.15 0.15 1.0]  GraphicEmissiveColor=[0.0 0.0 0.0 1.0]  GraphicShininess=75
  Gain : Gain  Gain=fcyl_len/max(max_fx,1e-3)
  Gain1 : Gain  Gain=-1
  Gain2 : Gain  Gain=fcyl_len/max(max_fy,1e-3)
  Gain3 : Gain  Gain=-1
  Gain4 : Gain  Gain=tcyl_rad/max(max_tz,1e-3)
  Gain5 : Gain  Gain=-1
  Saturation Fxn : Saturate  UpperLimit=inf  LowerLimit=0  ZeroCross=off
  Saturation Fxp : Saturate  UpperLimit=inf  LowerLimit=0  ZeroCross=off
  Saturation Fyn : Saturate  UpperLimit=inf  LowerLimit=0  ZeroCross=off
  Saturation Fyp : Saturate  UpperLimit=inf  LowerLimit=0  ZeroCross=off
  Saturation Tzn : Saturate  UpperLimit=inf  LowerLimit=0  ZeroCross=off
  Saturation Tzp : Saturate  UpperLimit=inf  LowerLimit=0  ZeroCross=off
  Simulink-PS Converter{1..6} (6 alike) : nesl_utility/Simulink-PS Converter  PhysicalDomain=network_engine_domain  SubClassName=ps_input  LeftPortType=input  RightPortType=output  PseudoPeriodic=off  Frequencies=[]  NoiseDistribution=none  NoiseParameters=[]  Unit=1  AffineConversion=off  FilteringAndDerivatives=provide  SimscapeFilterOrder=1  InputFilterTimeConstant=0.001  UdotUserProvided=0
  Transform cyl fxn : sm_lib/Frames and Transforms/Rigid Transform  RotationMethod=StandardAxis  FollAlignAxisA=+X  BaseAlignAxisA=+Y  FollAlignAxisB=+Y  BaseAlignAxisB=+Z  RotationStandardAxis=+Y  RotationAngle=-90  RotationAngleUnits=deg  RotationArbitraryAxis=[0 0 1]  RotationSequenceAxes=FollowerAxes  RotationSequence=XYX  RotationSequenceAngles=[0 0 0]  RotationSequenceAnglesUnits=deg  RotationMatrix=[1 0 0; 0 1 0; 0 0 1]  Quaternion=[1 0 0 0]  TranslationMethod=None  TranslationCartesianOffset=[0 0 0]  TranslationCartesianOffsetUnits=m  TranslationStandardAxis=+Z  TranslationStandardOffset=0  TranslationStandardOffsetUnits=m  TranslationROffset=0  TranslationROffsetUnits=m  TranslationThetaOffset=0  TranslationThetaOffsetUnits=deg  TranslationZOffset=0  TranslationZOffsetUnits=m
  Transform cyl fxp : sm_lib/Frames and Transforms/Rigid Transform  RotationMethod=StandardAxis  FollAlignAxisA=+X  BaseAlignAxisA=+Y  FollAlignAxisB=+Y  BaseAlignAxisB=+Z  RotationStandardAxis=+Y  RotationAngle=90  RotationAngleUnits=deg  RotationArbitraryAxis=[0 0 1]  RotationSequenceAxes=FollowerAxes  RotationSequence=XYX  RotationSequenceAngles=[0 0 0]  RotationSequenceAnglesUnits=deg  RotationMatrix=[1 0 0; 0 1 0; 0 0 1]  Quaternion=[1 0 0 0]  TranslationMethod=None  TranslationCartesianOffset=[0 0 0]  TranslationCartesianOffsetUnits=m  TranslationStandardAxis=+Z  TranslationStandardOffset=0  TranslationStandardOffsetUnits=m  TranslationROffset=0  TranslationROffsetUnits=m  TranslationThetaOffset=0  TranslationThetaOffsetUnits=deg  TranslationZOffset=0  TranslationZOffsetUnits=m
  Transform cyl fyn : sm_lib/Frames and Transforms/Rigid Transform  RotationMethod=StandardAxis  FollAlignAxisA=+X  BaseAlignAxisA=+Y  FollAlignAxisB=+Y  BaseAlignAxisB=+Z  RotationStandardAxis=+X  RotationAngle=90  RotationAngleUnits=deg  RotationArbitraryAxis=[0 0 1]  RotationSequenceAxes=FollowerAxes  RotationSequence=XYX  RotationSequenceAngles=[0 0 0]  RotationSequenceAnglesUnits=deg  RotationMatrix=[1 0 0; 0 1 0; 0 0 1]  Quaternion=[1 0 0 0]  TranslationMethod=None  TranslationCartesianOffset=[0 0 0]  TranslationCartesianOffsetUnits=m  TranslationStandardAxis=+Z  TranslationStandardOffset=0  TranslationStandardOffsetUnits=m  TranslationROffset=0  TranslationROffsetUnits=m  TranslationThetaOffset=0  TranslationThetaOffsetUnits=deg  TranslationZOffset=0  TranslationZOffsetUnits=m
  Transform cyl fyp : sm_lib/Frames and Transforms/Rigid Transform  RotationMethod=StandardAxis  FollAlignAxisA=+X  BaseAlignAxisA=+Y  FollAlignAxisB=+Y  BaseAlignAxisB=+Z  RotationStandardAxis=+X  RotationAngle=-90  RotationAngleUnits=deg  RotationArbitraryAxis=[0 0 1]  RotationSequenceAxes=FollowerAxes  RotationSequence=XYX  RotationSequenceAngles=[0 0 0]  RotationSequenceAnglesUnits=deg  RotationMatrix=[1 0 0; 0 1 0; 0 0 1]  Quaternion=[1 0 0 0]  TranslationMethod=None  TranslationCartesianOffset=[0 0 0]  TranslationCartesianOffsetUnits=m  TranslationStandardAxis=+Z  TranslationStandardOffset=0  TranslationStandardOffsetUnits=m  TranslationROffset=0  TranslationROffsetUnits=m  TranslationThetaOffset=0  TranslationThetaOffsetUnits=deg  TranslationZOffset=0  TranslationZOffsetUnits=m
  Transform cyl tzn : sm_lib/Frames and Transforms/Rigid Transform  RotationMethod=None  FollAlignAxisA=+X  BaseAlignAxisA=+Y  FollAlignAxisB=+Y  BaseAlignAxisB=+Z  RotationStandardAxis=+X  RotationAngle=90  RotationAngleUnits=deg  RotationArbitraryAxis=[0 0 1]  RotationSequenceAxes=FollowerAxes  RotationSequence=XYX  RotationSequenceAngles=[0 0 0]  RotationSequenceAnglesUnits=deg  RotationMatrix=[1 0 0; 0 1 0; 0 0 1]  Quaternion=[1 0 0 0]  TranslationMethod=None  TranslationCartesianOffset=[0 0 0]  TranslationCartesianOffsetUnits=m  TranslationStandardAxis=+Z  TranslationStandardOffset=0  TranslationStandardOffsetUnits=m  TranslationROffset=0  TranslationROffsetUnits=m  TranslationThetaOffset=0  TranslationThetaOffsetUnits=deg  TranslationZOffset=0  TranslationZOffsetUnits=m
  Transform cyl tzp : sm_lib/Frames and Transforms/Rigid Transform  RotationMethod=None  FollAlignAxisA=+X  BaseAlignAxisA=+Y  FollAlignAxisB=+Y  BaseAlignAxisB=+Z  RotationStandardAxis=+X  RotationAngle=-90  RotationAngleUnits=deg  RotationArbitraryAxis=[0 0 1]  RotationSequenceAxes=FollowerAxes  RotationSequence=XYX  RotationSequenceAngles=[0 0 0]  RotationSequenceAnglesUnits=deg  RotationMatrix=[1 0 0; 0 1 0; 0 0 1]  Quaternion=[1 0 0 0]  TranslationMethod=None  TranslationCartesianOffset=[0 0 0]  TranslationCartesianOffsetUnits=m  TranslationStandardAxis=+Z  TranslationStandardOffset=0  TranslationStandardOffsetUnits=m  TranslationROffset=0  TranslationROffsetUnits=m  TranslationThetaOffset=0  TranslationThetaOffsetUnits=deg  TranslationZOffset=0  TranslationZOffsetUnits=m
  R : PMIOPort  Side=Right
  wires:
  Bus Selector/1 -> Gain/1  "<fx>"
  Gain/1 -> Saturation Fxp/1, Gain1/1
  Saturation Fxp/1 -> Simulink-PS Converter6/1
  Gain1/1 -> Saturation Fxn/1
  Saturation Fxn/1 -> Simulink-PS Converter1/1
  Saturation Fyn/1 -> Simulink-PS Converter2/1
  Gain3/1 -> Saturation Fyn/1
  Saturation Fyp/1 -> Simulink-PS Converter3/1
  Gain2/1 -> Gain3/1, Saturation Fyp/1
  Bus Selector1/1 -> Gain2/1  "<fy>"
  T/1 -> Bus Selector2/1, Bus Selector1/1, Bus Selector/1
  Bus Selector2/1 -> Gain4/1  "<tz>"
  Gain4/1 -> Saturation Tzp/1, Gain5/1
  Saturation Tzp/1 -> Simulink-PS Converter5/1
  Gain5/1 -> Saturation Tzn/1
  Saturation Tzn/1 -> Simulink-PS Converter4/1
  connections:
  Cyl Tzn/LConn2 -- Cyl Fxn/LConn2 -- Cyl Mass/RConn1 -- Cyl Fxp/LConn2 -- Cyl Fyp/LConn2 -- Cyl Fyn/LConn2 -- Cyl Tzp/LConn2
  Simulink-PS Converter6/RConn1 -- Cyl Fxp/LConn1
  Transform cyl fxp/RConn1 -- Cyl Fxp/RConn1
  Transform cyl tzn/LConn1 -- R/RConn1 -- Transform cyl fxn/LConn1 -- Transform cyl fxp/LConn1 -- Transform cyl fyn/LConn1 -- Transform cyl fyp/LConn1 -- Transform cyl tzp/LConn1
  Transform cyl fxn/RConn1 -- Cyl Fxn/RConn1
  Cyl Fxn/LConn1 -- Simulink-PS Converter1/RConn1
  Cyl Fyn/LConn1 -- Simulink-PS Converter2/RConn1
  Transform cyl fyp/RConn1 -- Cyl Fyp/RConn1
  Simulink-PS Converter3/RConn1 -- Cyl Fyp/LConn1
  Transform cyl fyn/RConn1 -- Cyl Fyn/RConn1
  Transform cyl tzn/RConn1 -- Cyl Tzn/RConn1
  Simulink-PS Converter5/RConn1 -- Cyl Tzp/LConn1
  Cyl Tzn/LConn1 -- Simulink-PS Converter4/RConn1
  Transform cyl tzp/RConn1 -- Cyl Tzp/RConn1

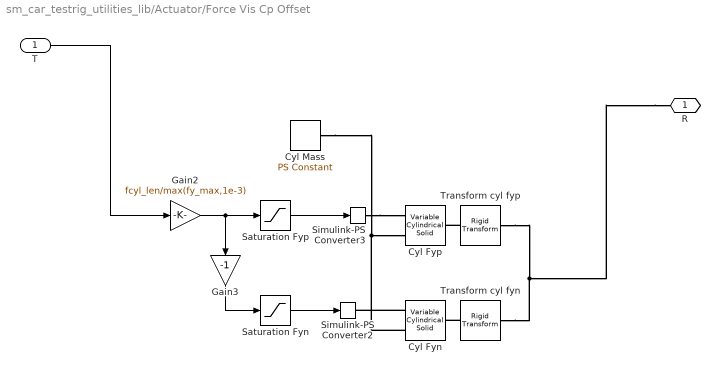
== system sm_car_testrig_utilities_lib/Actuator/Force Vis Cp Offset ==
  T : Inport
  Cyl Fyn : sm_lib/Body Elements/Variable Mass/Variable Cylindrical Solid  RadiusType=Constant  Radius=fcyl_rad  RadiusUnits=m  LengthType=ProvidedByInput  Length=1e-3  LengthUnits=m  MassType=ProvidedByInput  Density=1000  DensityUnits=kg/m^3  SenseRadius=off  SenseLength=off  SenseMass=off  SenseCenterOfMass=off  SenseInertiaMatrix=off  GraphicType=FromGeometry  MarkerShape=Sphere  MarkerSize=10  GraphicVisPropType=SimpleVisualProperties  GraphicDiffuseColor=fcyl_clr  GraphicOpacity=fcyl_opc  GraphicSpecularColor=[0.5 0.5 0.5 1.0]  GraphicAmbientColor=[0.15 0.15 0.15 1.0]  GraphicEmissiveColor=[0.0 0.0 0.0 1.0]  GraphicShininess=75
  Cyl Fyp : sm_lib/Body Elements/Variable Mass/Variable Cylindrical Solid  RadiusType=Constant  Radius=fcyl_rad  RadiusUnits=m  LengthType=ProvidedByInput  Length=1e-3  LengthUnits=m  MassType=ProvidedByInput  Density=1000  DensityUnits=kg/m^3  SenseRadius=off  SenseLength=off  SenseMass=off  SenseCenterOfMass=off  SenseInertiaMatrix=off  GraphicType=FromGeometry  MarkerShape=Sphere  MarkerSize=10  GraphicVisPropType=SimpleVisualProperties  GraphicDiffuseColor=fcyl_clr  GraphicOpacity=fcyl_opc  GraphicSpecularColor=[0.5 0.5 0.5 1.0]  GraphicAmbientColor=[0.15 0.15 0.15 1.0]  GraphicEmissiveColor=[0.0 0.0 0.0 1.0]  GraphicShininess=75
  Cyl Mass : fl_lib/Physical Signals/Sources/PS Constant  constant=1e-3
  Gain2 : Gain  Gain=fcyl_len/max(fy_max,1e-3)
  Gain3 : Gain  Gain=-1
  Saturation Fyn : Saturate  UpperLimit=inf  LowerLimit=0  ZeroCross=off
  Saturation Fyp : Saturate  UpperLimit=inf  LowerLimit=0  ZeroCross=off
  Simulink-PS Converter2 : nesl_utility/Simulink-PS Converter  PhysicalDomain=network_engine_domain  SubClassName=ps_input  LeftPortType=input  RightPortType=output  PseudoPeriodic=off  Frequencies=[]  NoiseDistribution=none  NoiseParameters=[]  Unit=1  AffineConversion=off  FilteringAndDerivatives=provide  SimscapeFilterOrder=1  InputFilterTimeConstant=0.001  UdotUserProvided=0
  Simulink-PS Converter3 : nesl_utility/Simulink-PS Converter  PhysicalDomain=network_engine_domain  SubClassName=ps_input  LeftPortType=input  RightPortType=output  PseudoPeriodic=off  Frequencies=[]  NoiseDistribution=none  NoiseParameters=[]  Unit=1  AffineConversion=off  FilteringAndDerivatives=provide  SimscapeFilterOrder=1  InputFilterTimeConstant=0.001  UdotUserProvided=0
  Transform cyl fyn : sm_lib/Frames and Transforms/Rigid Transform  RotationMethod=StandardAxis  FollAlignAxisA=+X  BaseAlignAxisA=+Y  FollAlignAxisB=+Y  BaseAlignAxisB=+Z  RotationStandardAxis=+X  RotationAngle=90  RotationAngleUnits=deg  RotationArbitraryAxis=[0 0 1]  RotationSequenceAxes=FollowerAxes  RotationSequence=XYX  RotationSequenceAngles=[0 0 0]  RotationSequenceAnglesUnits=deg  RotationMatrix=[1 0 0; 0 1 0; 0 0 1]  Quaternion=[1 0 0 0]  TranslationMethod=None  TranslationCartesianOffset=[0 0 0]  TranslationCartesianOffsetUnits=m  TranslationStandardAxis=+Z  TranslationStandardOffset=0  TranslationStandardOffsetUnits=m  TranslationROffset=0  TranslationROffsetUnits=m  TranslationThetaOffset=0  TranslationThetaOffsetUnits=deg  TranslationZOffset=0  TranslationZOffsetUnits=m
  Transform cyl fyp : sm_lib/Frames and Transforms/Rigid Transform  RotationMethod=StandardAxis  FollAlignAxisA=+X  BaseAlignAxisA=+Y  FollAlignAxisB=+Y  BaseAlignAxisB=+Z  RotationStandardAxis=+X  RotationAngle=-90  RotationAngleUnits=deg  RotationArbitraryAxis=[0 0 1]  RotationSequenceAxes=FollowerAxes  RotationSequence=XYX  RotationSequenceAngles=[0 0 0]  RotationSequenceAnglesUnits=deg  RotationMatrix=[1 0 0; 0 1 0; 0 0 1]  Quaternion=[1 0 0 0]  TranslationMethod=None  TranslationCartesianOffset=[0 0 0]  TranslationCartesianOffsetUnits=m  TranslationStandardAxis=+Z  TranslationStandardOffset=0  TranslationStandardOffsetUnits=m  TranslationROffset=0  TranslationROffsetUnits=m  TranslationThetaOffset=0  TranslationThetaOffsetUnits=deg  TranslationZOffset=0  TranslationZOffsetUnits=m
  R : PMIOPort  Side=Right
  wires:
  T/1 -> Gain2/1
  Gain2/1 -> Saturation Fyp/1, Gain3/1
  Saturation Fyp/1 -> Simulink-PS Converter3/1
  Gain3/1 -> Saturation Fyn/1
  Saturation Fyn/1 -> Simulink-PS Converter2/1
  connections:
  Transform cyl fyn/RConn1 -- Cyl Fyn/RConn1
  Simulink-PS Converter3/RConn1 -- Cyl Fyp/LConn1
  Transform cyl fyp/RConn1 -- Cyl Fyp/RConn1
  Cyl Fyn/LConn1 -- Simulink-PS Converter2/RConn1
  R/RConn1 -- Transform cyl fyp/LConn1 -- Transform cyl fyn/LConn1
  Cyl Fyn/LConn2 -- Cyl Mass/RConn1 -- Cyl Fyp/LConn2
